simulink model "ecu_injdur"  (R2026a)
settings: Solver=FixedStepDiscrete  StopTime=10  FixedStep=0.001  SampleTimeConstraint=STIndependent
Description:
  | Injector law, fitted to the old ECU (field evidence 2026-10-14 sec. 3d).
settings Model: Creator=jj1001000  LastModifiedBy=jj1001000
settings OptimizationCC: DefaultUnderspecifiedDataType=single
settings DebuggingCC: ParameterPrecisionLossMsg=none
settings HardwareCC: ProdLargestAtomicInteger=Long  ProdLargestAtomicFloat=Double  ProdHWDeviceType=ARM Compatible->ARM Cortex-M
settings RTWCC: SystemTargetFile=ert.tlc  GenCodeOnly=on  Description=Embedded Coder
settings ERTTargetCC: UtilityFuncGeneration=Shared location  IncludeMdlTerminateFcn=off  CodeInterfacePackaging=Reusable function  SupportNonFinite=off

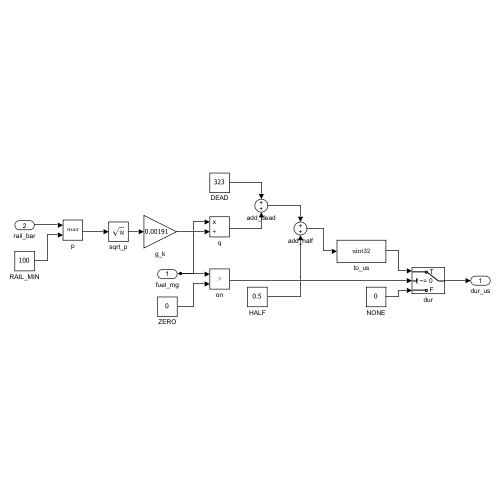
[thumbnail: Simulink's stored preview of the top-level diagram]
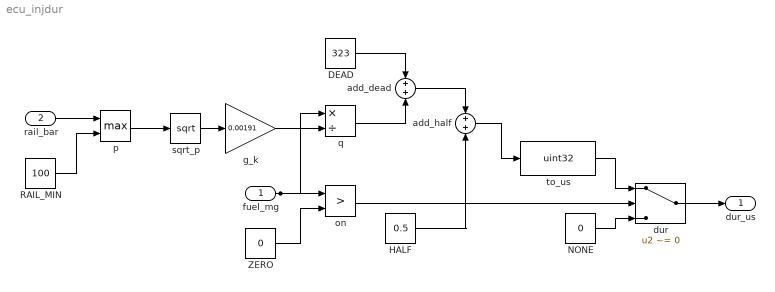
== system ecu_injdur ==
  fuel_mg : Inport  OutDataTypeStr=single
  rail_bar : Inport  Port=2  OutDataTypeStr=single
  DEAD : Constant  Value=323  OutDataTypeStr=single
  HALF : Constant  Value=0.5  OutDataTypeStr=single
  NONE : Constant  Value=0  OutDataTypeStr=uint32
  RAIL_MIN : Constant  Value=100  OutDataTypeStr=single
  ZERO : Constant  Value=0  OutDataTypeStr=single
  add_dead : Sum
  add_half : Sum
  dur : Switch  Criteria=u2 ~= 0  SaturateOnIntegerOverflow=off  InputSameDT=off
  g_k : Gain  Gain=0.00191
  on : RelationalOperator  Operator=>  OutDataTypeStr=boolean  RndMeth=Simplest  InputSameDT=off
  p : MinMax  Function=max  Inputs=2
  q : Product  Inputs=*/
  sqrt_p : Sqrt  OutDataTypeStr=single
  to_us : DataTypeConversion  OutDataTypeStr=uint32  SaturateOnIntegerOverflow=off
  dur_us : Outport  OutDataTypeStr=uint32
  wires:
  fuel_mg/1 -> on/1, q/1
  p/1 -> sqrt_p/1
  RAIL_MIN/1 -> p/2
  rail_bar/1 -> p/1
  DEAD/1 -> add_dead/1
  ZERO/1 -> on/2
  add_half/1 -> to_us/1
  HALF/1 -> add_half/2
  g_k/1 -> q/2
  sqrt_p/1 -> g_k/1
  add_dead/1 -> add_half/1
  q/1 -> add_dead/2
  on/1 -> dur/2
  to_us/1 -> dur/1
  NONE/1 -> dur/3
  dur/1 -> dur_us/1
